simulink model "ClarkeTransforms"  (R2026b)
settings: Solver=VariableStepAuto
settings Model: Creator=24322  LastModifiedBy=24322

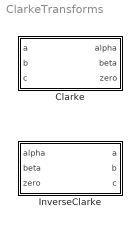
== system ClarkeTransforms ==
  Clarke : Subsystem
  InverseClarke : Subsystem

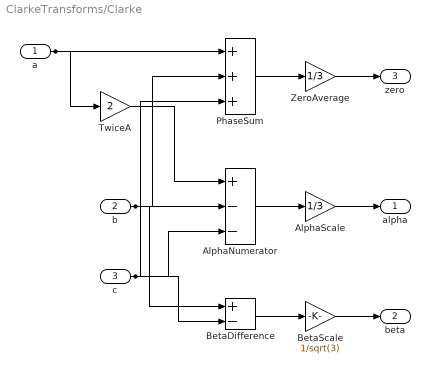
== system ClarkeTransforms/Clarke ==
  a : Inport  OutDataTypeStr=double
  b : Inport  Port=2  OutDataTypeStr=double
  c : Inport  Port=3  OutDataTypeStr=double
  AlphaNumerator : Sum  Inputs=+--
  AlphaScale : Gain  Gain=1/3
  BetaDifference : Sum  Inputs=+-
  BetaScale : Gain  Gain=1/sqrt(3)
  PhaseSum : Sum  Inputs=+++
  TwiceA : Gain  Gain=2
  ZeroAverage : Gain  Gain=1/3
  alpha : Outport
  beta : Outport  Port=2
  zero : Outport  Port=3
  wires:
  ZeroAverage/1 -> zero/1
  PhaseSum/1 -> ZeroAverage/1
  BetaScale/1 -> beta/1
  BetaDifference/1 -> BetaScale/1
  AlphaScale/1 -> alpha/1
  AlphaNumerator/1 -> AlphaScale/1
  c/1 -> BetaDifference/2, AlphaNumerator/3, PhaseSum/3
  b/1 -> BetaDifference/1, AlphaNumerator/2, PhaseSum/2
  TwiceA/1 -> AlphaNumerator/1
  a/1 -> PhaseSum/1, TwiceA/1

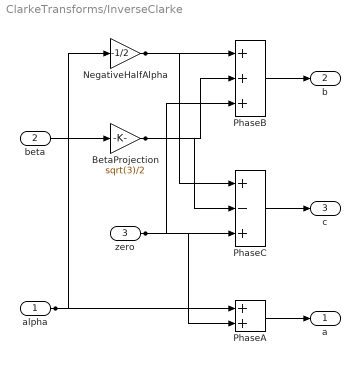
== system ClarkeTransforms/InverseClarke ==
  alpha : Inport  OutDataTypeStr=double
  beta : Inport  Port=2  OutDataTypeStr=double
  zero : Inport  Port=3  OutDataTypeStr=double
  BetaProjection : Gain  Gain=sqrt(3)/2
  NegativeHalfAlpha : Gain  Gain=-1/2
  PhaseA : Sum
  PhaseB : Sum  Inputs=+++
  PhaseC : Sum  Inputs=+-+
  a : Outport
  b : Outport  Port=2
  c : Outport  Port=3
  wires:
  PhaseC/1 -> c/1
  PhaseB/1 -> b/1
  PhaseA/1 -> a/1
  BetaProjection/1 -> PhaseB/2, PhaseC/2
  NegativeHalfAlpha/1 -> PhaseB/1, PhaseC/1
  zero/1 -> PhaseA/2, PhaseB/3, PhaseC/3
  beta/1 -> BetaProjection/1
  alpha/1 -> PhaseA/1, NegativeHalfAlpha/1
